simulink model "sfRectifyAPIExample"  (R2025b)
settings: Solver=VariableStepAuto  StartTime=0.0  StopTime=10.0  RelTol=1e-3
settings Model: Creator=The MathWorks, Inc.  LastModifiedBy=The MathWorks, Inc.
settings OptimizationCC: ReuseModelBlockBuffer=off
settings RTWCC: GPUComputeCapability=3.5

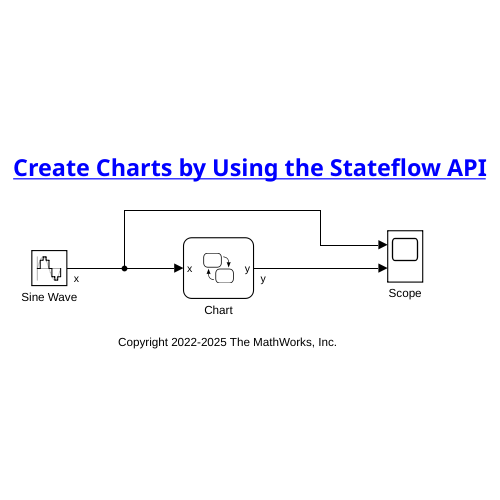
[thumbnail: Simulink's stored preview of the top-level diagram]
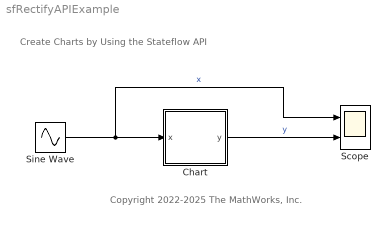
== system sfRectifyAPIExample ==
  note: Copyright 2022-2025 The MathWorks, Inc.
  note: Create Charts by Using the Stateflow API
  Chart : Stateflow chart  TreatAsAtomicUnit=on
  Scope : Scope  NumInputPorts=2
      settings: ActiveDisplayYMinimum=-1.24563  ActiveDisplayYMaximum=1.24904
  Sine Wave : Sin  SampleTime=0.2
  wires:
  Sine Wave/1 -> Scope/1, Chart/1(x)  "x"
  Chart/1(y) -> Scope/2  "y"

== stateflow chart sfRectifyAPIExample/Chart ==
  state On
    y = x;
  state Off
    y = 0;
  (default) -> On
  On -> Off : [x<t0]
  Off -> On : [x>=t0]
  data: x input double; y output single; t0 constant fixdt(1,5,2) =0
